simulink model "Quadrotor_aerial_load_wind_effect"  (R2024a)
settings: Solver=FixedStepAuto  StartTime=0.0  StopTime=50  FixedStep=0.01  MaxStep=0.0001  MinStep=0.00001  RelTol=1e-9
undefined symbols (not defined in the file): F, Light, MIL
libraries: aerolibwind2 x1
settings Model: Creator=salor  LastModifiedBy=aarl0
settings SolverCC: AlgebraicLoopSolver=TrustRegion
settings DataIOCC: ReturnWorkspaceOutputs=off
settings DebuggingCC: UnconnectedInputMsg=warning  UnconnectedOutputMsg=warning  UnconnectedLineMsg=warning  ArithmeticOperatorsInVariantConditions=warning
settings ModelReferenceCC: EnableRefExpFcnMdlSchedulingChecks=on
settings SFSimCC: SimUseLocalCustomCode=off  CustomCodeUndefinedFunction=UseInterfaceOnly
settings RTWCC: RTWUseLocalCustomCode=off  GPUComputeCapability=3.5
settings CodeAppCC: StateflowObjectComments=on

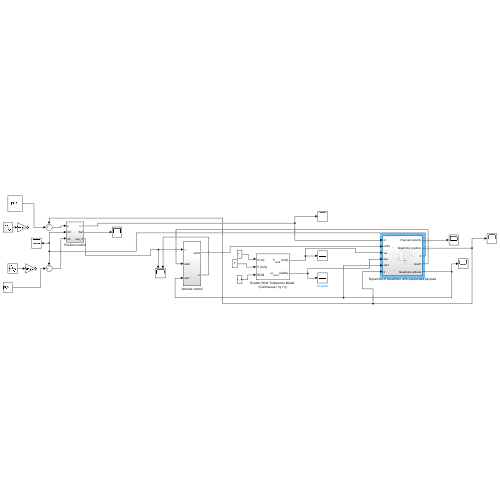
[thumbnail: Simulink's stored preview of the top-level diagram]
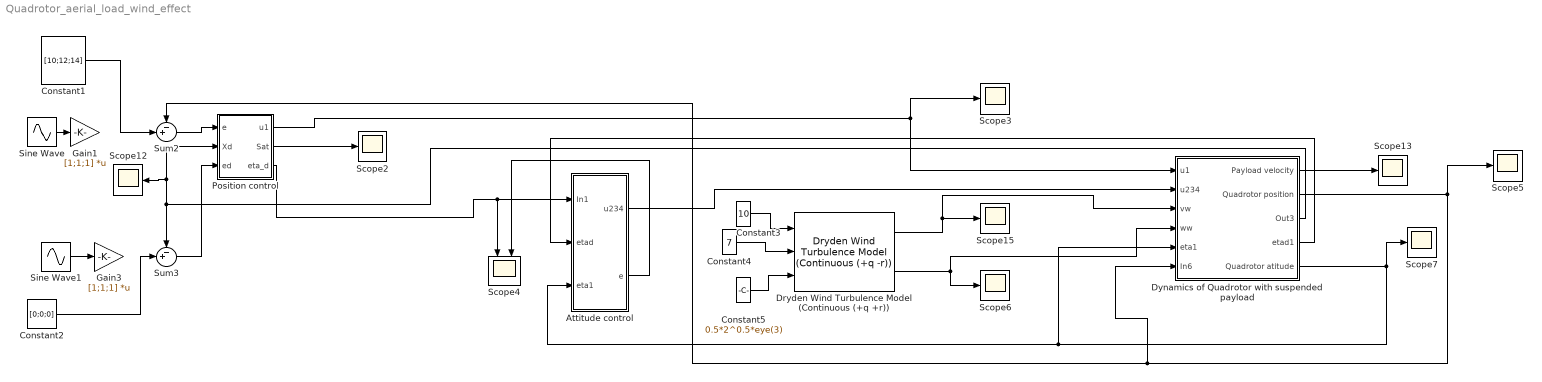
== system Quadrotor_aerial_load_wind_effect ==
  Attitude control : Subsystem
  Constant1 : Constant  Value=[10;12;14]
  Constant2 : Constant  Value=[0;0;0]
  Constant3 : Constant  Value=10
  Constant4 : Constant  Value=7
  Constant5 : Constant  Value=0.5*2^0.5*eye(3)
  Dryden Wind Turbulence Model (Continuous (+q +r)) : aerolibwind2/Dryden Wind Turbulence Model  (Continuous (+q -r))  units=Metric (MKS)  spec=MIL-F-8785C  model=Continuous Dryden (+q +r)  W20=15  Wdeg=0  TurbProb=10^-2 - Light  L_high=533.4  Wingspan=10  ts=0.1  Seed=[23341 23342 23343 23344]  T_on=on
  Dynamics of Quadrotor with suspended payload : Subsystem
  Gain1 : Gain  Gain=[1;1;1]  Multiplication=Matrix(K*u) (u vector)
  Gain3 : Gain  Gain=[1;1;1]  Multiplication=Matrix(K*u) (u vector)
  Position control : Subsystem
  Scope{2..3,5..7,12..13,15} (8 alike) : Scope
  Scope4 : Scope  NumInputPorts=2
  Sine Wave : Sin  Amplitude=0.1  Bias=10  Frequency=.4*pi  SampleTime=0
  Sine Wave1 : Sin  Amplitude=pi*0.04  Frequency=.4*pi  Phase=pi/2  SampleTime=0
  Sum2 : Sum  Inputs=-+|
  Sum3 : Sum  Inputs=-+|
  wires:
  Sine Wave/1 -> Gain1/1
  Sine Wave1/1 -> Gain3/1
  Constant1/1 -> Sum2/2
  Constant2/1 -> Sum3/2
  Dryden Wind Turbulence Model (Continuous (+q +r))/1 -> Dynamics of Quadrotor with suspended payload/3(vw), Scope15/1
  Dryden Wind Turbulence Model (Continuous (+q +r))/2 -> Dynamics of Quadrotor with suspended payload/4(ww), Scope6/1
  Constant3/1 -> Dryden Wind Turbulence Model (Continuous (+q +r))/1
  Constant5/1 -> Dryden Wind Turbulence Model (Continuous (+q +r))/3
  Constant4/1 -> Dryden Wind Turbulence Model (Continuous (+q +r))/2
  Position control/1(u1) -> Dynamics of Quadrotor with suspended payload/1(u1), Scope3/1
  Position control/3(eta_d) -> Scope4/1, Attitude control/1(In1)
  Sum2/1 -> Position control/1(e)
  Sum3/1 -> Position control/3(ed)
  Position control/2(Sat) -> Scope2/1
  Attitude control/2(e) -> Scope4/2
  Dynamics of Quadrotor with suspended payload/3(Out3) -> Position control/2(Xd), Scope12/1, Sum3/1
  Dynamics of Quadrotor with suspended payload/2(Quadrotor position) -> Scope5/1, Dynamics of Quadrotor with suspended payload/6(In6), Sum2/1
  Dynamics of Quadrotor with suspended payload/5(Quadrotor atitude) -> Scope7/1, Dynamics of Quadrotor with suspended payload/5(eta1), Attitude control/3(eta1)
  Attitude control/1(u234) -> Dynamics of Quadrotor with suspended payload/2(u234)
  Dynamics of Quadrotor with suspended payload/1(Payload velocity) -> Scope13/1
  Dynamics of Quadrotor with suspended payload/4(etad1) -> Attitude control/2(etad)

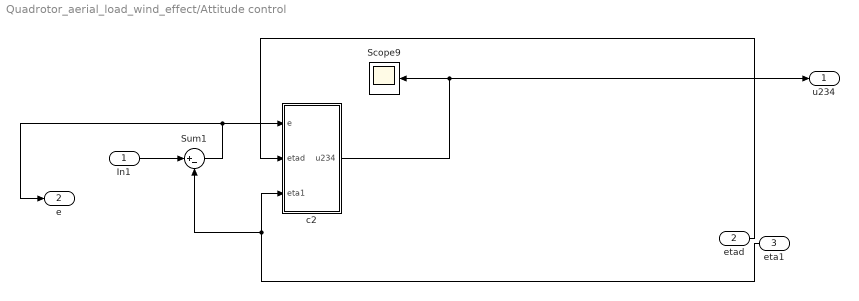
== system Quadrotor_aerial_load_wind_effect/Attitude control ==
  In1 : Inport
  etad : Inport  Port=2
  eta1 : Inport  Port=3
  Scope9 : Scope
  Sum1 : Sum  Inputs=|+-
  c2 : MATLAB Function  TreatAsAtomicUnit=on
  u234 : Outport
  e : Outport  Port=2
  wires:
  c2/1(u234) -> u234/1, Scope9/1
  Sum1/1 -> e/1, c2/1(e)
  eta1/1 -> Sum1/2, c2/3(eta1)
  In1/1 -> Sum1/1
  etad/1 -> c2/2(etad)

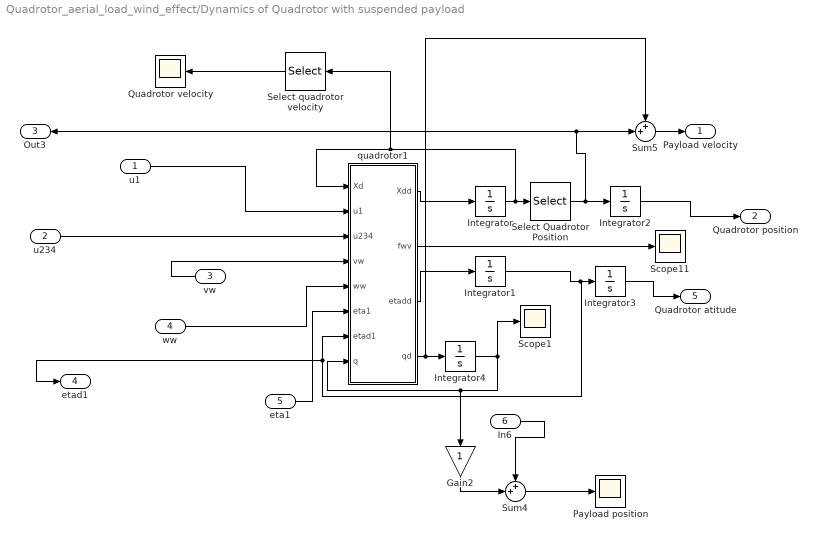
== system Quadrotor_aerial_load_wind_effect/Dynamics of Quadrotor with suspended payload ==
  u1 : Inport
  u234 : Inport  Port=2
  vw : Inport  Port=3
  ww : Inport  Port=4
  eta1 : Inport  Port=5
  In6 : Inport  Port=6
  Gain2 : Gain
  Integrator : Integrator  InitialCondition=[0;0;0;0;0;0]
  Integrator1 : Integrator  InitialCondition=[0;0;0]
  Integrator2 : Integrator  InitialCondition=[0;1;2]
  Integrator3 : Integrator  InitialCondition=[pi/60;pi/40;pi/60]
  Integrator4 : Integrator  InitialCondition=[0;0;1]
  Payload position : Scope
  Quadrotor velocity : Scope
  Scope1 : Scope
  Scope11 : Scope
  Select Quadrotor Position : Selector  InputPortWidth=6  IndexOptions=Index vector (dialog)  Indices=[1:3]  OutputSizes=1
  Select quadrotor velocity : Selector  InputPortWidth=6  IndexOptions=Index vector (dialog)  Indices=[4:6]  OutputSizes=1
  Sum4 : Sum  Inputs=++|
  Sum5 : Sum  Inputs=++|
  quadrotor1 : MATLAB Function  TreatAsAtomicUnit=on
  Payload velocity : Outport
  Quadrotor position : Outport  Port=2
  Out3 : Outport  Port=3
  etad1 : Outport  Port=4
  Quadrotor atitude : Outport  Port=5
  wires:
  Integrator1/1 -> etad1/1, quadrotor1/7(etad1), Integrator3/1
  ww/1 -> quadrotor1/5(ww)
  Select Quadrotor Position/1 -> Integrator2/1, Out3/1, Sum5/2
  Select quadrotor velocity/1 -> Quadrotor velocity/1
  vw/1 -> quadrotor1/4(vw)
  quadrotor1/3(etadd) -> Integrator1/1
  Integrator/1 -> Select quadrotor velocity/1, quadrotor1/1(Xd), Select Quadrotor Position/1
  quadrotor1/4(qd) -> Integrator4/1, Sum5/1
  Sum4/1 -> Payload position/1
  In6/1 -> Sum4/1
  quadrotor1/1(Xdd) -> Integrator/1
  Gain2/1 -> Sum4/2
  quadrotor1/2(fwv) -> Scope11/1
  Integrator4/1 -> quadrotor1/8(q), Gain2/1, Scope1/1
  Integrator3/1 -> Quadrotor atitude/1
  Integrator2/1 -> Quadrotor position/1
  Sum5/1 -> Payload velocity/1
  eta1/1 -> quadrotor1/6(eta1)
  u1/1 -> quadrotor1/2(u1)
  u234/1 -> quadrotor1/3(u234)

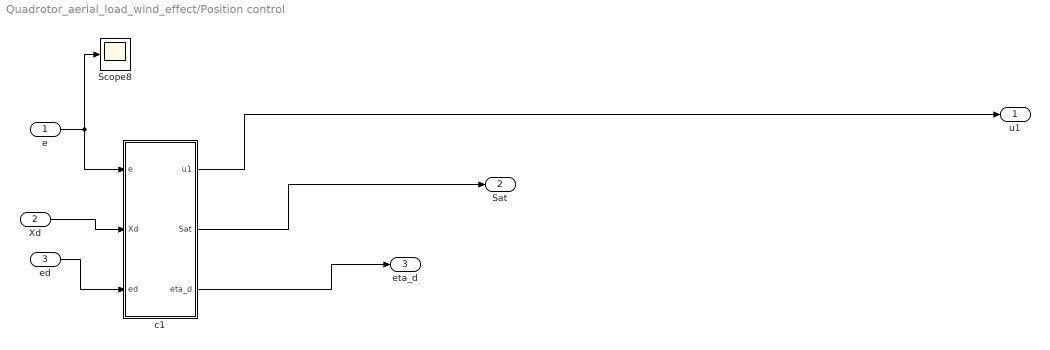
== system Quadrotor_aerial_load_wind_effect/Position control ==
  e : Inport
  Xd : Inport  Port=2
  ed : Inport  Port=3
  Scope8 : Scope
  c1 : MATLAB Function  TreatAsAtomicUnit=on
  u1 : Outport
  Sat : Outport  Port=2
  eta_d : Outport  Port=3
  wires:
  e/1 -> Scope8/1, c1/1(e)
  c1/3(eta_d) -> eta_d/1
  c1/1(u1) -> u1/1
  Xd/1 -> c1/2(Xd)
  ed/1 -> c1/3(ed)
  c1/2(Sat) -> Sat/1

== matlab function Quadrotor_aerial_load_wind_effect/Position control/c1 ==
  data: e input; Xd input; u1 output; Sat output; ed input; eta_d output
function [u1,Sat,eta_d]   = fcn(e,Xd,ed)
% fi=eta1(1);teta=eta1(2);sai=eta1(3);
% fid=etad1(1);tetad=etad1(2);said=etad1(3);
g=9.81;%Ix=7.5*10^-3; Iy=7.5*10^-3;
% Iz=1.3*10^-2;Jr=6.5*10^-5;b=3.13*10^-5;
% l=0.23;
m=0.775;k1=diag([25 25 0.01]);k2=1*k1;

% a1=(Iy-Iz)/Ix; a2=Jr/Ix; a3=(Iz-Ix)/Iy; a4=Jr/Iy;
% a5=(Ix-Iy)/Iz; b1=l/Ix; b2=l/Iy; b3=l/Iz;
u=k1*e+k2*ed+[0;0;-g];
% if u(3)<g
%     u(3)=0;
% end
kp=diag([0.1 0.1 0.1]);
a=sqrt(2/3);bh=diag([a a a]);
fhw=(3-2)/2*ones(3,1);fhp=1.5*ones(3,1);ep1=.008;ep2=.008;ep3=0.008;
landa=01*diag([0.76;.6;.8]);M=01.5*diag([10 10 16]);
S=landa*e+ed;
if S(1)>ep1
    st1=1;
 elseif S(1)<-ep1
    st1=-1;
 else
     st1=S(1)/ep2;
end
if S(2)>ep2
    st2=1;
 elseif S(2)<-ep2
    st2=-1;
 else
     st2=S(2)/ep2;
end
if S(3)>ep2
    st3=1;
 elseif S(3)<-ep3
    st3=-1;
 else
     st3=S(3)/ep3;
end

Sat=[st1;st2;st3];
u=inv(bh)*(-fhw+fhp+kp*Xd(1:3)-landa*ed-M*Sat)+[0;0;g];
uu=sqrt(u'*u);
teta_d1=atan(-u(1)/(u(3)-g));
fi_d1=atan(-(u(2)*cos(teta_d1))/(g-u(3)));
u1=u(3)/(cos(fi_d1)*cos(teta_d1));
eta_d=[fi_d1;teta_d1;0];
% et=angdiff(eta_d,eta);
end

== matlab function Quadrotor_aerial_load_wind_effect/Attitude control/c2 ==
  data: u234 output; e input; etad input; eta1 input
function u234  = fcn(e,etad,eta1)
 fi1=eta1(1);teta1=eta1(2);sai=eta1(3);z=4;
% % fid=etad(1);tetad=etad(2);said=etad1(3);
% g=9.81;Ix=7.5*10^-3; Iy=7.5*10^-3;
% Iz=1.3*10^-2;Jr=6.5*10^-5;b=3.13*10^-5;
% l=0.23;m=1;

% o1=real(sqrt(complex(u1/(4*b)+u3/(2*b)-u4/(4*b))));
% o2=real(s
m=1;K1=.50;K2=0.10;k=5;g=9.81;
% u1=-m*(-g+K1*(z-Xq3))/(cos(fi1)*cos(teta1));

e1_q1=e(1);e1_q2=e(2);e1_q3=e(3);
fid1=etad(1);tetad1=etad(2);said1=etad(3);
u2=K1*(e1_q1)-K2*fid1;
u3=K1*(e1_q2)-K2*tetad1;
u4=K1*(e1_q3)-K2*said1;
u234=[u2;u3;u4];
end

== matlab function Quadrotor_aerial_load_wind_effect/Dynamics of Quadrotor with suspended payload/quadrotor1 ==
  data: Xd input; u1 input; Xdd output; fwv output; u234 input; vw input; ww input; eta1 input; etad1 input; etadd output; q input; qd output
function [Xdd,fwv,etadd,qd] = fcn(Xd,u1,u234,vw,ww,eta1,etad1,q)
fi=eta1(1);teta=eta1(2);sai=eta1(3);
fid=etad1(1);tetad=etad1(2);said=etad1(3);
g=9.81;Ix=7.5*10^-3; Iy=7.5*10^-3;
Iz=1.3*10^-2;Jr=6.5*10^-5;b=3.13*10^-5;
bb=0.23;mq=0.775;ml=0.5;l=01;
VmXd=vw-Xd(1:3);wmXd=ww-Xd(4:6);
u2=u234(1);u3=u234(2);u4=u234(3);
o1=(sqrt(abs(u1/(4*b)+u3/(2*b)-u4/(4*b))));
o2=(sqrt(abs(u1/(4*b)-u2/(2*b)+u4/(4*b))));
o3=(sqrt(abs(u1/(4*b)-u3/(2*b)-u4/(4*b))));
o4=(sqrt(abs(u1/(4*b)+u2/(2*b)+u4/(4*b))));
omegar=o2+o4-o1-o3; 
a1=(Iy-Iz)/Ix; a2=Jr/Ix; a3=(Iz-Ix)/Iy; a4=Jr/Iy;
a5=(Ix-Iy)/Iz; b1=bb/Ix; b2=bb/Iy; b3=bb/Iz;
w=Xd(4:6)
mt=mq+ml;qh=[0 -q(3) q(2)
             q(3) 0 -q(1)
            -q(2) q(1) 0];e3=[0;0;1];
wh=[0 -w(3) w(2)
    w(3) 0 -w(1)
    -w(2) w(1) 0];
ro=1.22;C_dA=diag([0.05;0.05;0.1]);
kp=diag([0.1 0.1 0.1]);kr=0.12;
fww=0.5*ro*C_dA*(diag(wmXd))^2*sign(wmXd);
f1=tetad*said*a1-tetad*a2*omegar+b1*u2-kr*bb*fid/Ix;
f2=fid*said*a3+fid*a4*omegar+b2*u3-kr*bb*tetad/Iy;
f3=fid*tetad*a5+b3*u4-kr*bb*said/Iz;
etadd=([f1;f2;f3]);


fwv=0.5*ro*C_dA*(diag(VmXd))^2*sign(VmXd);
C_s=cos(sai);S_s=sin(sai);C_f=cos(fi);S_f=sin(fi);
C_t=cos(teta);S_t=sin(teta);
nw=norm(w);
R= [C_s*C_t       C_s*S_t*S_f-S_s*C_f    C_s*S_t*C_f+S_s*S_f
      S_s*C_t     C_s*C_f+S_s*S_t*S_f    S_s*S_t*C_f-C_s*S_f
        -S_t            C_t*S_f                C_t*C_f]; 
M=[mt*eye(3) -ml*l*qh;
    ml*l*qh  ml*l^2*eye(3)];
T=[fwv-kp*Xd(1:3)+mt*g*e3+ml*l*nw^2*q-u1*R*e3
    ml*g*l*qh*e3];
Xdd=inv(M)*(T);
qd=wh*q;
end
